simulink model "Lab2_VM_Task_1234_Testing"  (R2026a)
settings: Solver=FixedStepDiscrete  StopTime=Inf  FixedStep=0.02  EnableMultiTasking=on
undefined symbols (not defined in the file or in its folder): Angular, Linear
libraries: robotlib x3
settings Model: Creator=The MathWorks, Inc.  LastModifiedBy=juulg
settings OptimizationCC: LifeSpan=Inf
settings HardwareCC: ProdHWDeviceType=Generic->Unspecified (assume 32-bit Generic)  TargetHWDeviceType=Generic->Unspecified (assume 32-bit Generic)  UseEmbeddedCoderFeatures=off
settings SFSimCC: SimTargetLang=C++
settings RTWCC: SystemTargetFile=ert.tlc  HardwareBoard=Robot Operating System (ROS)  Toolchain=Catkin  TargetLang=C++  Description=Embedded Coder
settings ERTTargetCC: RootIOFormat=Structure reference  DynamicArrayContainerType=coder::array  MultiwordLength=2048.0  ERTCustomFileBanners=off  CodeInterfacePackaging=C++ class  SubcomponentCodeInterfacePackaging=C++ class  SupportContinuousTime=on  SupportNonInlinedSFcns=on  SupportVariableSizeSignals=on  ModelStepFunctionPrototypeControlCompliant=off

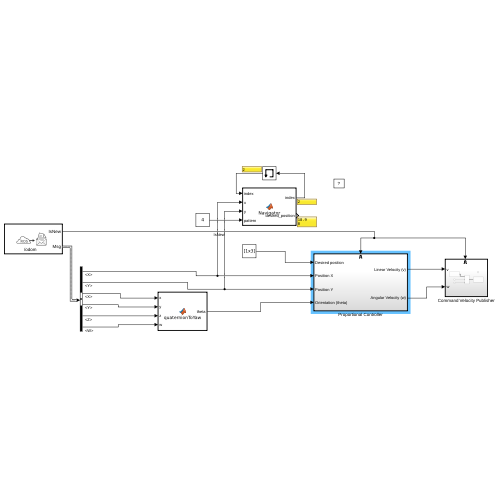
[thumbnail: Simulink's stored preview of the top-level diagram]
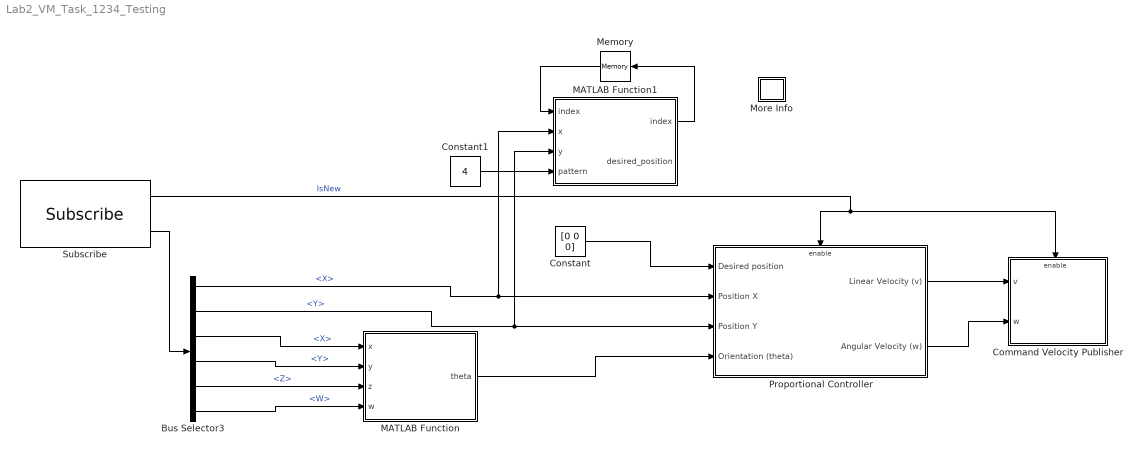
== system Lab2_VM_Task_1234_Testing ==
  Bus Selector3 : BusSelector  OutputSignals=Pose.Pose.Position.X,Pose.Pose.Position.Y,Pose.Pose.Orientation.X,Pose.Pose.Orientation.Y,Pose.Pose.Orientation.Z,Pose.Pose.Orientation.W
  Command Velocity Publisher : Subsystem
  Constant : Constant  Value=[0 0 0]  VectorParams1D=off
  Constant1 : Constant  Value=4
  MATLAB Function : MATLAB Function  TreatAsAtomicUnit=on
  MATLAB Function1 : MATLAB Function  TreatAsAtomicUnit=on
  Memory : Memory  InitialCondition=1
  More Info : Subsystem
      settings: OpenFcn=showdemo(bdroot(gcb))
      mask Display: disp('?')
  Proportional Controller : Subsystem
  Subscribe : robotlib/Subscribe  topicSource=Select from ROS network  topic=/odom  messageType=nav_msgs/Odometry  SampleTime=-1  legacyBusStruct=off  messageQueueLength=51
  wires:
  Subscribe/2 -> Bus Selector3/1
  Proportional Controller/1(Linear Velocity (v)) -> Command Velocity Publisher/1(v)
  Subscribe/1 -> Command Velocity Publisher/Enable, Proportional Controller/Enable  "IsNew"
  Bus Selector3/4 -> MATLAB Function/2(y)  "<Y>"
  Proportional Controller/2(Angular Velocity (w)) -> Command Velocity Publisher/2(w)
  Bus Selector3/2 -> MATLAB Function1/3(y), Proportional Controller/3(Position Y)  "<Y>"
  Bus Selector3/1 -> MATLAB Function1/2(x), Proportional Controller/2(Position X)  "<X>"
  MATLAB Function/1(theta) -> Proportional Controller/4(Orientation (theta))
  Bus Selector3/6 -> MATLAB Function/4(w)  "<W>"
  Bus Selector3/5 -> MATLAB Function/3(z)  "<Z>"
  Bus Selector3/3 -> MATLAB Function/1(x)  "<X>"
  MATLAB Function1/1(index) -> Memory/1
  Memory/1 -> MATLAB Function1/1("index ")
  Constant1/1 -> MATLAB Function1/4(pattern)
  Constant/1 -> Proportional Controller/1(Desired position)

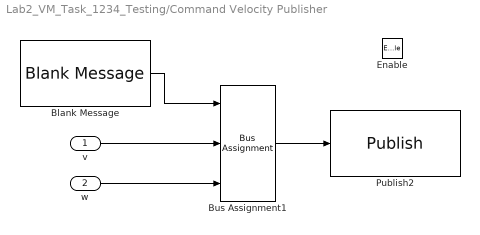
== system Lab2_VM_Task_1234_Testing/Command Velocity Publisher ==
  v : Inport
  w : Inport  Port=2
  Enable : EnablePort
  Blank Message : robotlib/Blank Message  messageClass=Message  entityType=geometry_msgs/Twist  messageType=geometry_msgs/Twist  SampleTime=inf  legacyBusStruct=off
  Bus Assignment1 : BusAssignment  DialogController=Simulink.DDGSource_BusAssignment  AssignedSignals=Linear.X,Angular.Z
  Publish2 : robotlib/Publish  topicSource=Select from ROS network  topic=/cmd_vel  messageType=geometry_msgs/Twist  legacyBusStruct=off  messageQueueLength=105
  wires:
  Bus Assignment1/1 -> Publish2/1
  Blank Message/1 -> Bus Assignment1/1
  v/1 -> Bus Assignment1/2
  w/1 -> Bus Assignment1/3

== system Lab2_VM_Task_1234_Testing/More Info ==

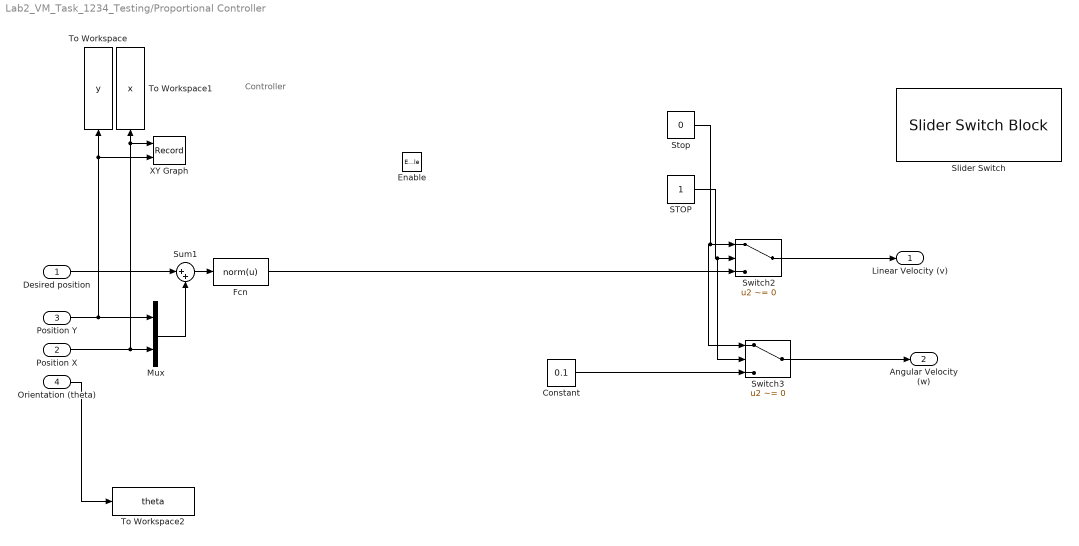
== system Lab2_VM_Task_1234_Testing/Proportional Controller ==
  note: Controller
  Desired position : Inport
  Position X : Inport  Port=2
  Position Y : Inport  Port=3
  Orientation (theta) : Inport  Port=4
  Enable : EnablePort
  Constant : Constant  Value=0.1
  Fcn : Fcn  Expr=norm(u)
  Mux : Mux  Inputs=2
  "STOP " : Constant
  Slider Switch : SliderSwitchBlock
  Stop : Constant  Value=0
  Sum1 : Sum  Inputs=|++
  Switch2 : Switch  Criteria=u2 ~= 0  SaturateOnIntegerOverflow=off  InputSameDT=off
  Switch3 : Switch  Criteria=u2 ~= 0  SaturateOnIntegerOverflow=off  InputSameDT=off
  To Workspace : ToWorkspace  VariableName=y  SaveFormat=Timeseries  SampleTime=-1
  To Workspace1 : ToWorkspace  VariableName=x  SaveFormat=Timeseries  SampleTime=-1
  To Workspace2 : ToWorkspace  VariableName=theta  SaveFormat=Timeseries  SampleTime=-1
  XY Graph : Record  NumPorts=2.0  FileSettingsInternal="{\"entries\":[{\"content\":{\"excelSettings\":{\"content\":{},\"type\":\"Streamout.ExcelSettings\"},\"parquetSettings\":{\"content\":{},\"type\":\"Streamout.ParquetSettings\"}},\"type\":\"Streamout.FileSettingStorage\",\"uuid\":\"\"}],\"packageUris\":[\"http:\\/\\/schema.mathworks.com\\/mf0\\/streamout_blocks\\/R2020a\"],\"version\":\"1.0\"}"  FrameSettings=[0, 0]  Layout=[1 1]  SignalsInternal="{\"entries\":[{\"content\":{\"signals\":[{\"content\":{\"blockPath\":[],\"dimensions\":[1],\"domain\":\"\",\"lineColor\":\"#a2142f\",\"plots\":[ 1 ],\"port\":1,\"sid\":[\"\"],\"signalID\":1,\"signalName\":\"X\"},\"type\":\"RecordBlkView.Signal\",\"uuid\":\"\"},{\"content\":{\"blockPath\":[],\"dimensions\":[1],\"domain\":\"\",\"lineColor\":\"#139fff\",\"plots\":[ 1 ],\"port\":2,\"sid\":[\"\"],\"signalID\":2,\"signalName\":\"Y\"},\"type\":\"RecordBlkView.Signal\",\"uuid\":\"\"}]},\"type\":\"RecordBlkView.InputSignals\",\"uuid\":\"\"}],\"packageUris\":[\"http:\\/\\/schema.mathworks.com\\/mf0\\/streamout_blocks\\/R2020a\"],\"version\":\"1.0\"}"  VisualizationBindings="{\"xyplotplugin\":{\"info\":[{\"series\":[{\"bindingParametersList\":[{\"parameter\":\"X-Axis\",\"signalID\":1,\"signalName\":\"X\"},{\"parameter\":\"Y-Axis\",\"signalID\":2,\"signalName\":\"Y\"}],\"seriesID\":0}],\"subplotID\":1}]}}"  CompatibilityTag=XY
  Linear Velocity (v) : Outport  VectorParamsAs1DForOutWhenUnconnected=off
  Angular Velocity (w) : Outport  Port=2  VectorParamsAs1DForOutWhenUnconnected=off
  wires:
  Stop/1 -> Switch3/1, Switch2/1
  "STOP "/1 -> Switch3/2, Switch2/2
  Switch2/1 -> Linear Velocity (v)/1
  Switch3/1 -> Angular Velocity (w)/1
  Orientation (theta)/1 -> To Workspace2/1
  Position X/1 -> Mux/2, To Workspace1/1, XY Graph/1
  Position Y/1 -> Mux/1, To Workspace/1, XY Graph/2
  Constant/1 -> Switch3/3
  Fcn/1 -> Switch2/3
  Desired position/1 -> Sum1/1
  Mux/1 -> Sum1/2
  Sum1/1 -> Fcn/1

== matlab function Lab2_VM_Task_1234_Testing/MATLAB Function1 ==
  data: index output; index input; desired_position output; x input; y input; pattern input
function [index,desired_position] = Navigator(index, x,y, pattern)
    square_motion = [0 10; 10 10; 10 0; 0 0];
    j_motion = [
    0 0;
    5.6533 0;
    5.6533 -8.1659;
    3.3501 -9.4221;
    0.8375 -9.2128;
    0 -7.3283
    ];
    i = linspace(0,360,20).';
    sin_motion = [i/9, 10*sin(deg2rad(i))];
    straight_motion=[i,zeros(1, length(i))'];
    % Store paths in a cell array
    patterns = {square_motion, j_motion, sin_motion, straight_motion};

    % Select current path
    current_pattern = patterns{pattern};

    % Get current waypoint
    desired_position = current_pattern(index,:);

    % Check distance to waypoint
    if norm(desired_position(1:2) - [x y]) < 0.12

        index = mod(index, size(current_pattern,1)) + 1;

        % Update desired waypoint
        desired_position = current_pattern(index,:);
    end
end

== matlab function Lab2_VM_Task_1234_Testing/MATLAB Function ==
  data: x input; theta output; y input; z input; w input
function theta = quaternionToYaw(x,y,z,w)

    theta = atan2(2*(w*z + x*y), ...
                  1 - 2*(y*y + z*z));

end
